simulink model "Bidirection_EVSE_V2G_and_G2V"  (R2024b)
settings: Solver=VariableStepAuto  StartTime=0.0  StopTime=10.0  RelTol=1e-3
undefined symbols (not defined in the file): Ion, Lithium
libraries: spsIdealSwitchLib x6, spsSeriesRLCBranchLib x6, slpidlib x4, spsPWMGeneratorDCDCLib x4, spsMosfetLib x4, spsVoltageMeasurementLib x4, spsThreePhaseSeriesRLCLoadLib x3, spsThreePhaseVIMeasurementLib x2, spsUniversalBridgeLib x2, spsBatteryLib x1, spsPLL3phLib x1, spsPower3phInstantaneousLib x1
settings Model: Creator=SUDHAK1  LastModifiedBy=SUDHAK1

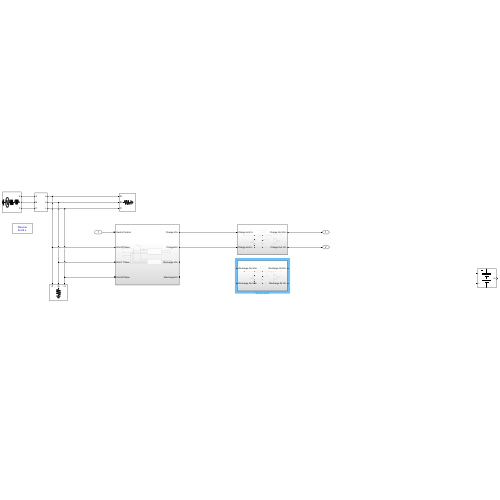
[thumbnail: Simulink's stored preview of the top-level diagram]
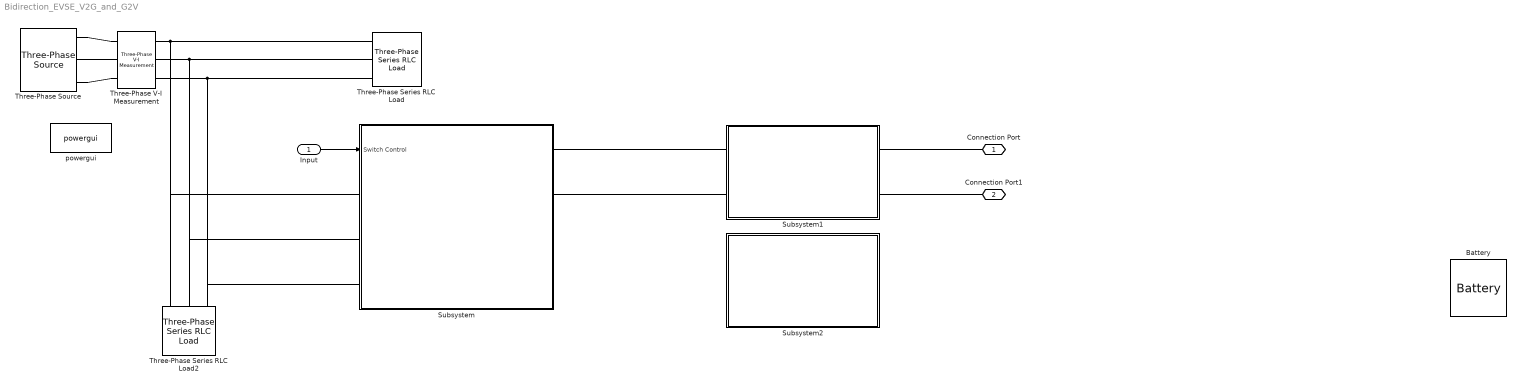
== system Bidirection_EVSE_V2G_and_G2V ==
  Input : Inport
  Battery : spsBatteryLib/Battery  BatType=Lithium-Ion  NomV=230  NomQ=100  SOC=60  Batt_Tr=1e-3  PresetModel=on  MaxQ=100  MinV=172.5  FullV=267.717  Dis_rate=43.4783  R=0.023  Normal_OP=90.4348  expZone="[248.4887      4.913043]"
  Subsystem : Subsystem
  Subsystem1 : Subsystem
  Subsystem2 : Subsystem
  Three-Phase Series RLC Load : spsThreePhaseSeriesRLCLoadLib/Three-Phase Series RLC Load  LConnTagsString=A|B|C  Configuration=Y (grounded)  NominalVoltage=380  Vabc=[1e3 1e3 1e3]  Vabcp=[1e3 1e3 1e3]  NominalFrequency=50  UnbalancedPower=off  ActivePower=10e3  InductivePower=0  CapacitivePower=0  Pabc=[10e3 9e3 11e3]  QLabc=[100 90 110]  QCabc=[100 90 110]  Pabcp=[10e3 9e3 11e3]  QLabcp=[100 90 110]  QCabcp=[100 90 110]  Measurements=None  LoadType=constant Z
  Three-Phase Series RLC Load2 : spsThreePhaseSeriesRLCLoadLib/Three-Phase Series RLC Load  LConnTagsString=A|B|C  Configuration=Y (grounded)  NominalVoltage=380  Vabc=[1e3 1e3 1e3]  Vabcp=[1e3 1e3 1e3]  NominalFrequency=50  UnbalancedPower=off  ActivePower=10e3  InductivePower=0  CapacitivePower=0  Pabc=[10e3 9e3 11e3]  QLabc=[100 90 110]  QCabc=[100 90 110]  Pabcp=[10e3 9e3 11e3]  QLabcp=[100 90 110]  QCabcp=[100 90 110]  Measurements=None  LoadType=constant Z
  Three-Phase V-I Measurement : spsThreePhaseVIMeasurementLib/Three-Phase V-I Measurement  VoltageMeasurement=phase-to-phase  SetLabelV=on  LabelV=Vabc_grid  Vpu=off  VpuLL=off  CurrentMeasurement=yes  SetLabelI=on  LabelI=Iabc_grid  Ipu=off  Pbase=100e6  Vbase=500e3  OutputType=Complex  PhasorSimulation=off  PSBequivalent=0
  Three-Phase Source : spsThreePhaseSourceLib/Three-Phase Source  InternalConnection=Yg  VoltagePhases=off  Voltage=380  PhaseAngle=0  Voltage_phases=[25e3 25e3 25e3]/sqrt(3)  PhaseAngles_phases=[0 -120 +120]  Frequency=50  NonIdealSource=on  SpecifyImpedance=on  Resistance=0.8929  Inductance=16.58e-3  ShortCircuitLevel=100e6  BaseVoltage=380  XRratio=7  BusType=swing  Pref=10e3  Qref=0  Prefabc=[10e3, 10e3, 10e3]  Qrefabc=[0, 0, 0]  Qmin=-inf  Qmax=inf
  powergui : spspowerguiLib/powergui  Priority=1  SimulationMode=Discrete  SampleTime=5e-6  frequency=60  Iterations=50  frequencyindice=60  Pbase=100e6  ErrMax=1e-4  UnitsV=kV  UnitsW=MW  buscounter=0  FunctionMessages=off  echomessages=off  EnableUseOfTLC=off  CurrentSourceSwitches=off  DisableSnubberDevices=off  DisableRonSwitches=off  DisableVfSwitches=off  DisplayEquations=off  AutomaticDiscreteSolvers=off  SolverType=Tustin/Backward Euler (TBE)  Interpol=off  ExternalGateDelay=off  methode=off  Ts=100  x0status=blocks  SPID=on  SwTol=0  HookPort=off  NonlinearTolerance=1e-4  nMaxIteration=100  ContinueOnMaxIteration=off  RestoreLinks=warning  ResistiveCurrentMeasurement=off  Frange=[0:2:500]  Ylog=off  Xlog=on  ShowGrid=off  save=off  variable=ZData  structure=0  ZoomFFT=off  StartTime=0.0  cycles=1  DisplayStyle=1  fundamental=60  FreqAxis=off  MaxFrequency=1000  frequencyindicesteady=1  RmsSteady=1  display=off
  Connection Port : PMIOPort  Side=Left
  Connection Port1 : PMIOPort  Port=2  Side=Left
  wires:
  Input/1 -> Subsystem/1(Switch Control)
  connections:
  Three-Phase Source/RConn1 -- Three-Phase V-I Measurement/LConn1
  Three-Phase Source/RConn2 -- Three-Phase V-I Measurement/LConn2
  Three-Phase Source/RConn3 -- Three-Phase V-I Measurement/LConn3
  Three-Phase Series RLC Load/LConn1 -- Three-Phase Series RLC Load2/LConn1 -- Subsystem/LConn1 -- Three-Phase V-I Measurement/RConn1
  Three-Phase Series RLC Load/LConn2 -- Three-Phase Series RLC Load2/LConn2 -- Subsystem/LConn2 -- Three-Phase V-I Measurement/RConn2
  Three-Phase Series RLC Load/LConn3 -- Three-Phase Series RLC Load2/LConn3 -- Subsystem/LConn3 -- Three-Phase V-I Measurement/RConn3
  Subsystem/RConn1 -- Subsystem1/LConn1
  Connection Port/RConn1 -- Subsystem1/RConn1
  Subsystem/RConn2 -- Subsystem1/LConn2
  Connection Port1/RConn1 -- Subsystem1/RConn2

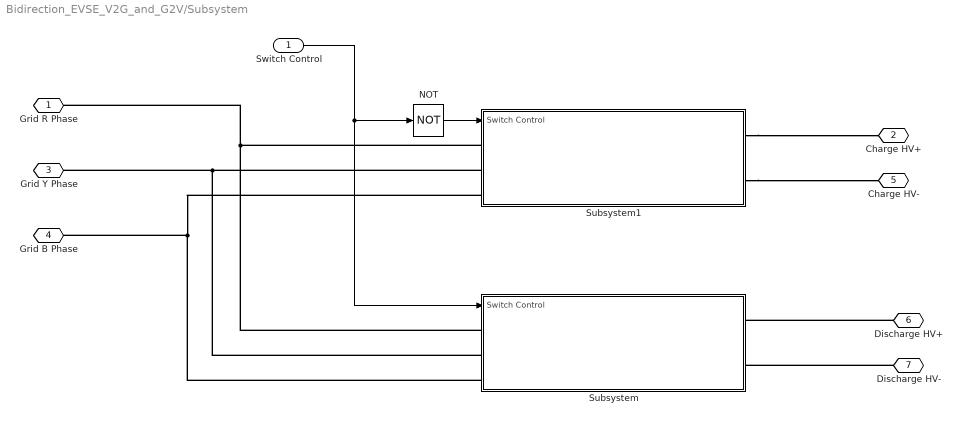
== system Bidirection_EVSE_V2G_and_G2V/Subsystem ==
  Switch Control : Inport
  NOT : Logic  Operator=NOT  IconShape=distinctive  AllPortsSameDT=off  OutDataTypeStr=boolean
  Subsystem : Subsystem
  Subsystem1 : Subsystem
  Grid R Phase : PMIOPort  Side=Left
  Charge HV+ : PMIOPort  Port=2  Side=Right
  Grid Y Phase : PMIOPort  Port=3  Side=Left
  Grid B Phase : PMIOPort  Port=4  Side=Left
  Charge HV- : PMIOPort  Port=5  Side=Right
  Discharge HV+ : PMIOPort  Port=6  Side=Right
  Discharge HV- : PMIOPort  Port=7  Side=Right
  wires:
  Switch Control/1 -> Subsystem/1(Switch Control), NOT/1
  NOT/1 -> Subsystem1/1(Switch Control)
  connections:
  Subsystem/LConn2 -- Grid Y Phase/RConn1 -- Subsystem1/LConn2
  Grid B Phase/RConn1 -- Subsystem1/LConn3 -- Subsystem/LConn3
  Subsystem/LConn1 -- Grid R Phase/RConn1 -- Subsystem1/LConn1
  Subsystem1/RConn1 -- Charge HV+/RConn1
  Subsystem1/RConn2 -- Charge HV-/RConn1
  Discharge HV-/RConn1 -- Subsystem/RConn2
  Discharge HV+/RConn1 -- Subsystem/RConn1

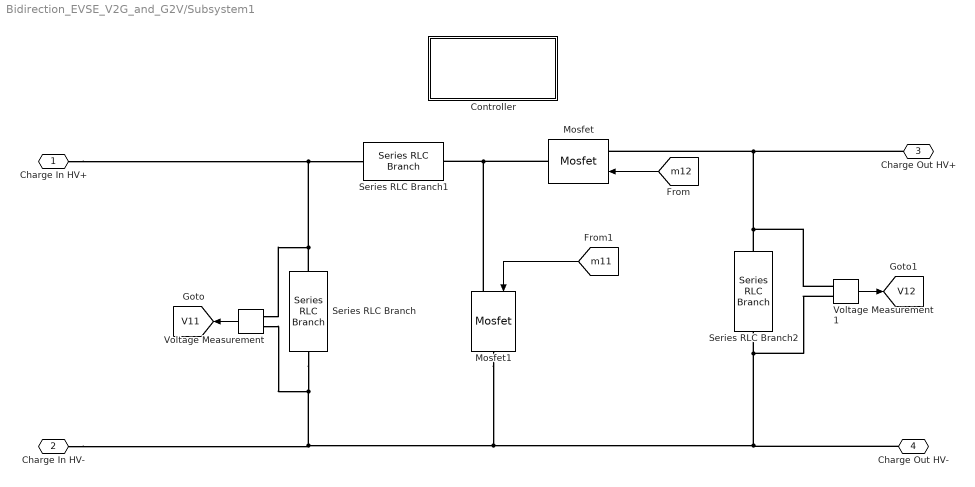
== system Bidirection_EVSE_V2G_and_G2V/Subsystem1 ==
  Controller : Subsystem
  Mosfet : spsMosfetLib/Mosfet  Ron=0.1  Lon=0  Rd=0.01  Vfd=0  IC=0  Rs=1e5  Cs=inf  Measurements=off
  Mosfet1 : spsMosfetLib/Mosfet  Ron=0.1  Lon=0  Rd=0.01  Vfd=0  IC=0  Rs=1e5  Cs=inf  Measurements=off
  Series RLC Branch : spsSeriesRLCBranchLib/Series RLC Branch  LConnTagsString=__new0  RConnTagsString=__new0  BranchType=RC  Resistance=0.0001  Inductance=1e-3  SetiL0=off  InitialCurrent=0  Capacitance=1000e-6  Setx0=off  InitialVoltage=0  Measurements=None
  Series RLC Branch1 : spsSeriesRLCBranchLib/Series RLC Branch  LConnTagsString=__new0  RConnTagsString=__new0  BranchType=L  Resistance=0.0001  Inductance=1e-3  SetiL0=off  InitialCurrent=0  Capacitance=1000e-6  Setx0=off  InitialVoltage=0  Measurements=None
  Series RLC Branch2 : spsSeriesRLCBranchLib/Series RLC Branch  LConnTagsString=__new0  RConnTagsString=__new0  BranchType=RC  Resistance=0.0001  Inductance=1e-3  SetiL0=off  InitialCurrent=0  Capacitance=1000e-6  Setx0=off  InitialVoltage=0  Measurements=None
  Voltage Measurement : spsVoltageMeasurementLib/Voltage Measurement  PhasorSimulation=off  OutputType=Complex  PSBequivalent=0
  Voltage Measurement1 : spsVoltageMeasurementLib/Voltage Measurement  PhasorSimulation=off  OutputType=Complex  PSBequivalent=0
  Charge In HV+ : PMIOPort  Side=Left
  Charge In HV- : PMIOPort  Port=2  Side=Left
  Charge Out HV+ : PMIOPort  Port=3  Side=Right
  Charge Out HV- : PMIOPort  Port=4  Side=Right
  tag scope: V11=global, V12=global
  wires:
  Voltage Measurement1/1 -> [V12]
  Voltage Measurement/1 -> [V11]
  [m11] -> Mosfet1/1
  [m12] -> Mosfet/1
  connections:
  Series RLC Branch/RConn1 -- Charge In HV-/RConn1 -- Mosfet1/RConn1 -- Charge Out HV-/RConn1 -- Voltage Measurement1/LConn2 -- Series RLC Branch2/RConn1 -- Voltage Measurement/LConn2
  Voltage Measurement/LConn1 -- Charge In HV+/RConn1 -- Series RLC Branch1/LConn1 -- Series RLC Branch/LConn1
  Series RLC Branch2/LConn1 -- Voltage Measurement1/LConn1 -- Charge Out HV+/RConn1 -- Mosfet/LConn1
  Mosfet/RConn1 -- Mosfet1/LConn1 -- Series RLC Branch1/RConn1

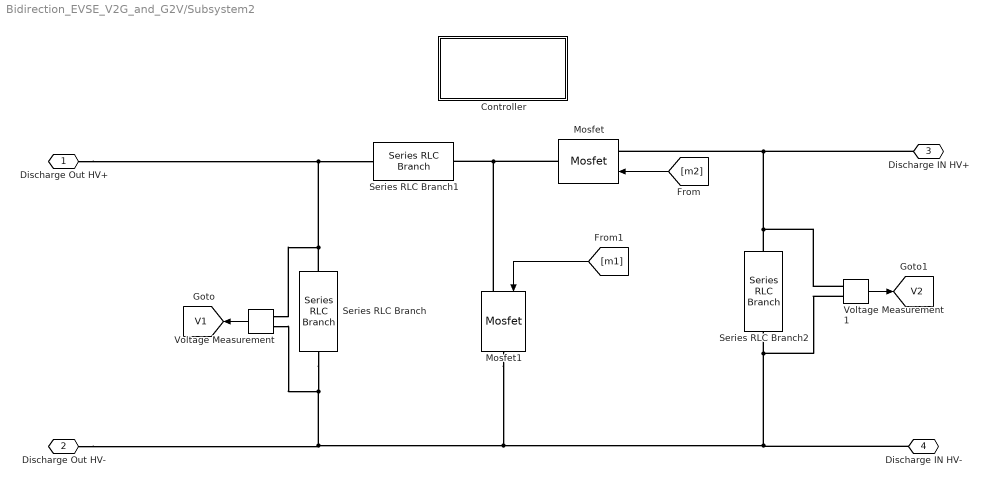
== system Bidirection_EVSE_V2G_and_G2V/Subsystem2 ==
  Controller : Subsystem
  Mosfet : spsMosfetLib/Mosfet  Ron=0.1  Lon=0  Rd=0.01  Vfd=0  IC=0  Rs=1e5  Cs=inf  Measurements=off
  Mosfet1 : spsMosfetLib/Mosfet  Ron=0.1  Lon=0  Rd=0.01  Vfd=0  IC=0  Rs=1e5  Cs=inf  Measurements=off
  Series RLC Branch : spsSeriesRLCBranchLib/Series RLC Branch  LConnTagsString=__new0  RConnTagsString=__new0  BranchType=RC  Resistance=0.0001  Inductance=1e-3  SetiL0=off  InitialCurrent=0  Capacitance=1000e-6  Setx0=off  InitialVoltage=0  Measurements=None
  Series RLC Branch1 : spsSeriesRLCBranchLib/Series RLC Branch  LConnTagsString=__new0  RConnTagsString=__new0  BranchType=L  Resistance=0.0001  Inductance=1e-3  SetiL0=off  InitialCurrent=0  Capacitance=1000e-6  Setx0=off  InitialVoltage=0  Measurements=None
  Series RLC Branch2 : spsSeriesRLCBranchLib/Series RLC Branch  LConnTagsString=__new0  RConnTagsString=__new0  BranchType=RC  Resistance=0.0001  Inductance=1e-3  SetiL0=off  InitialCurrent=0  Capacitance=1000e-6  Setx0=off  InitialVoltage=0  Measurements=None
  Voltage Measurement : spsVoltageMeasurementLib/Voltage Measurement  PhasorSimulation=off  OutputType=Complex  PSBequivalent=0
  Voltage Measurement1 : spsVoltageMeasurementLib/Voltage Measurement  PhasorSimulation=off  OutputType=Complex  PSBequivalent=0
  Discharge Out HV+ : PMIOPort  Side=Left
  Discharge Out HV- : PMIOPort  Port=2  Side=Left
  Discharge IN HV+ : PMIOPort  Port=3  Side=Right
  Discharge IN HV- : PMIOPort  Port=4  Side=Right
  tag scope: V1=global, V2=global
  wires:
  Voltage Measurement1/1 -> [V2]
  Voltage Measurement/1 -> [V1]
  [m1] -> Mosfet1/1
  [m2] -> Mosfet/1
  connections:
  Series RLC Branch/RConn1 -- Voltage Measurement/LConn2 -- Discharge Out HV-/RConn1 -- Mosfet1/RConn1 -- Discharge IN HV-/RConn1 -- Voltage Measurement1/LConn2 -- Series RLC Branch2/RConn1
  Voltage Measurement/LConn1 -- Series RLC Branch/LConn1 -- Series RLC Branch1/LConn1 -- Discharge Out HV+/RConn1
  Voltage Measurement1/LConn1 -- Series RLC Branch2/LConn1 -- Discharge IN HV+/RConn1 -- Mosfet/LConn1
  Mosfet/RConn1 -- Series RLC Branch1/RConn1 -- Mosfet1/LConn1

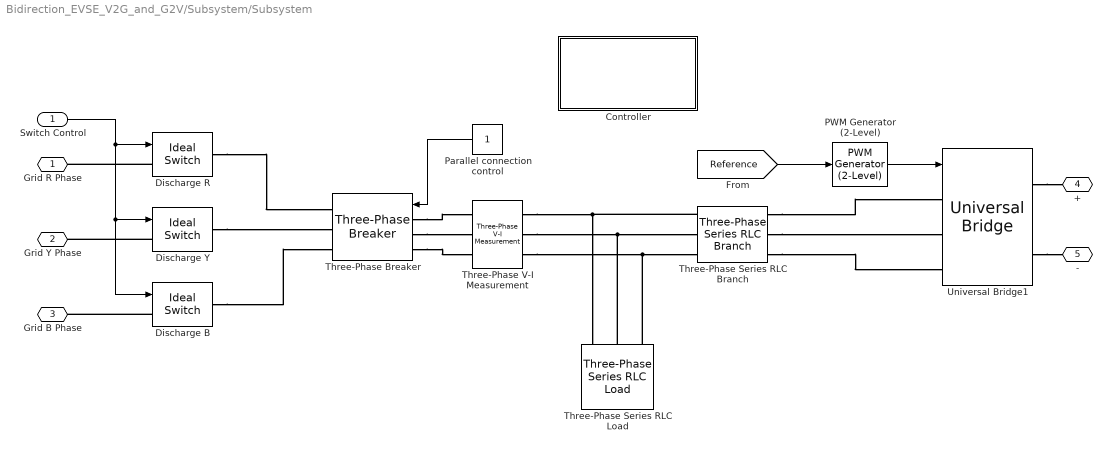
== system Bidirection_EVSE_V2G_and_G2V/Subsystem/Subsystem ==
  Switch Control : Inport
  Controller : Subsystem
  Discharge B : spsIdealSwitchLib/Ideal Switch  Ron=1e-6  Lon=0  IC=0  Rs=1e5  Cs=inf  Measurements=off
  Discharge R : spsIdealSwitchLib/Ideal Switch  Ron=1e-6  Lon=0  IC=0  Rs=1e5  Cs=inf  Measurements=off
  Discharge Y : spsIdealSwitchLib/Ideal Switch  Ron=1e-6  Lon=0  IC=0  Rs=1e5  Cs=inf  Measurements=off
  PWM Generator (2-Level) : spsPWMGenerator2LevelLib/PWM Generator (2-Level)  ModulatorType=Three-phase bridge (6 pulses)  ModulatorMode=Unsynchronized  Fc=4950  Pc=90  nF=27  MinMax="[ -1  1 ]"  SamplingTechnique=Natural  ModulatingSignals=off  m=0.8  Freq=60  Phase=0  Ts=2.02e-6  ShowCarrierOutport=off
  Parallel connection control : Constant
  Three-Phase Series RLC Branch : spsThreePhaseSeriesRLCBranchLib/Three-Phase Series RLC Branch  LConnTagsString=A|B|C  RConnTagsString=A|B|C  BranchType=RL  Resistance=0.004332  Inductance=0.0013789184  Capacitance=1e-6  Measurements=None
  Three-Phase Series RLC Load : spsThreePhaseSeriesRLCLoadLib/Three-Phase Series RLC Load  LConnTagsString=A|B|C  Configuration=Delta  NominalVoltage=380  Vabc=[1e3 1e3 1e3]  Vabcp=[1e3 1e3 1e3]  NominalFrequency=50  UnbalancedPower=off  ActivePower=100  InductivePower=0  CapacitivePower=5000  Pabc=[10e3 9e3 11e3]  QLabc=[100 90 110]  QCabc=[100 90 110]  Pabcp=[10e3 9e3 11e3]  QLabcp=[100 90 110]  QCabcp=[100 90 110]  Measurements=None  LoadType=constant Z
  Three-Phase V-I Measurement : spsThreePhaseVIMeasurementLib/Three-Phase V-I Measurement  VoltageMeasurement=phase-to-phase  SetLabelV=on  LabelV=Vabc_inv  Vpu=off  VpuLL=off  CurrentMeasurement=yes  SetLabelI=on  LabelI=Iabc_inv  Ipu=off  Pbase=100e6  Vbase=500e3  OutputType=Complex  PhasorSimulation=off  PSBequivalent=0
  Three-Phase Breaker : spsThreePhaseBreakerLib/Three-Phase Breaker  InitialState=open  SwitchA=on  SwitchB=on  SwitchC=on  SwitchTimes="[1/60  5/60]"  External=on  BreakerResistance=0.01  SnubberResistance=1e6  SnubberCapacitance=inf  Measurements=None
  Universal Bridge1 : spsUniversalBridgeLib/Universal Bridge  Arms=3  SnubberResistance=1e6  SnubberCapacitance=inf  Device=IGBT / Diodes  Ron=1e-3  Lon=0  ForwardVoltages="[  0  0  ]"  ForwardVoltage=0  GTOparameters=[ 10e-6 , 20e-6 ]  IGBTparameters=[ 1e-6 , 2e-6 ]  Measurements=None  Measurements_2=None  converterType=Rectifier
  Grid R Phase : PMIOPort  Side=Left
  Grid Y Phase : PMIOPort  Port=2  Side=Left
  Grid B Phase : PMIOPort  Port=3  Side=Left
  + : PMIOPort  Port=4  Side=Right
  - : PMIOPort  Port=5  Side=Right
  wires:
  [Reference] -> PWM Generator (2-Level)/1
  PWM Generator (2-Level)/1 -> Universal Bridge1/1
  Switch Control/1 -> Discharge B/1, Discharge Y/1, Discharge R/1
  Parallel connection control/1 -> Three-Phase Breaker/1
  connections:
  Three-Phase Series RLC Branch/LConn3 -- Universal Bridge1/LConn3
  Three-Phase Breaker/LConn1 -- Three-Phase V-I Measurement/RConn1
  Three-Phase Series RLC Branch/RConn1 -- Three-Phase Series RLC Load/LConn1 -- Three-Phase V-I Measurement/LConn1
  Three-Phase Breaker/LConn2 -- Three-Phase V-I Measurement/RConn2
  Discharge B/RConn1 -- Three-Phase Breaker/RConn3
  Discharge Y/RConn1 -- Three-Phase Breaker/RConn2
  Three-Phase Breaker/LConn3 -- Three-Phase V-I Measurement/RConn3
  Discharge R/RConn1 -- Three-Phase Breaker/RConn1
  Three-Phase Series RLC Load/LConn3 -- Three-Phase V-I Measurement/LConn3 -- Three-Phase Series RLC Branch/RConn3
  Three-Phase Series RLC Load/LConn2 -- Three-Phase V-I Measurement/LConn2 -- Three-Phase Series RLC Branch/RConn2
  Discharge B/LConn1 -- Grid B Phase/RConn1
  Three-Phase Series RLC Branch/LConn1 -- Universal Bridge1/LConn1
  Three-Phase Series RLC Branch/LConn2 -- Universal Bridge1/LConn2
  Discharge R/LConn1 -- Grid R Phase/RConn1
  Universal Bridge1/RConn2 -- -/RConn1
  Discharge Y/LConn1 -- Grid Y Phase/RConn1
  Universal Bridge1/RConn1 -- +/RConn1

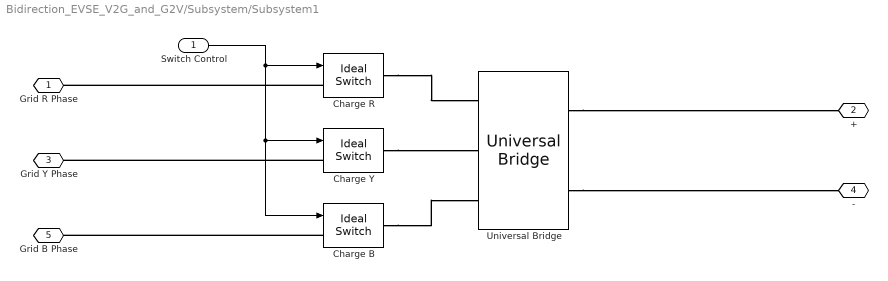
== system Bidirection_EVSE_V2G_and_G2V/Subsystem/Subsystem1 ==
  Switch Control : Inport
  Charge B : spsIdealSwitchLib/Ideal Switch  Ron=1e-6  Lon=0  IC=0  Rs=1e5  Cs=inf  Measurements=off
  Charge R : spsIdealSwitchLib/Ideal Switch  Ron=1e-6  Lon=0  IC=0  Rs=1e5  Cs=inf  Measurements=off
  Charge Y : spsIdealSwitchLib/Ideal Switch  Ron=1e-6  Lon=0  IC=0  Rs=1e5  Cs=inf  Measurements=off
  Universal Bridge : spsUniversalBridgeLib/Universal Bridge  Arms=3  SnubberResistance=1e5  SnubberCapacitance=inf  Device=Diodes  Ron=1e-3  Lon=0  ForwardVoltages="[  0  0  ]"  ForwardVoltage=0  GTOparameters=[ 10e-6 , 20e-6 ]  IGBTparameters=[ 1e-6 , 2e-6 ]  Measurements=None  Measurements_2=None  converterType=Rectifier
  Grid R Phase : PMIOPort  Side=Left
  + : PMIOPort  Port=2  Side=Right
  Grid Y Phase : PMIOPort  Port=3  Side=Left
  - : PMIOPort  Port=4  Side=Right
  Grid B Phase : PMIOPort  Port=5  Side=Left
  wires:
  Switch Control/1 -> Charge Y/1, Charge B/1, Charge R/1
  connections:
  Charge B/LConn1 -- Grid B Phase/RConn1
  Universal Bridge/RConn1 -- +/RConn1
  Charge B/RConn1 -- Universal Bridge/LConn3
  Charge R/RConn1 -- Universal Bridge/LConn1
  Charge R/LConn1 -- Grid R Phase/RConn1
  Charge Y/RConn1 -- Universal Bridge/LConn2
  Charge Y/LConn1 -- Grid Y Phase/RConn1
  Universal Bridge/RConn2 -- -/RConn1

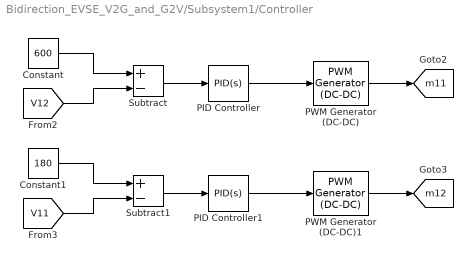
== system Bidirection_EVSE_V2G_and_G2V/Subsystem1/Controller ==
  Constant : Constant  Value=600
  Constant1 : Constant  Value=180
  PID Controller : slpidlib/PID Controller  Controller=PID  Form=Parallel  TimeDomain=Continuous-time  UseExternalTs=off  SampleTime=-1  IntegratorMethod=Forward Euler  FilterMethod=Forward Euler  ControllerParametersSource=internal  P=0  I=7  UseKiTs=off  D=0  UseExternalDerivativeSource=off  N=100  UseFilter=on  TunerSelectOption=Transfer Function Based (PID Tuner App)  InitialConditionSource=internal  InitialConditionForIntegrator=0  InitialConditionForFilter=0  DifferentiatorICPrevScaledInput=0  ExternalReset=none  TrackingMode=off  Kt=1  LimitOutput=off  SatLimitsSource=internal  UpperSaturationLimit=inf  LowerSaturationLimit=-inf  LinearizeAsGain=on  AntiWindupMode=none  Kb=1  LimitIntegrator=off  UpperIntegratorSaturationLimit=inf  LowerIntegratorSaturationLimit=-inf  POutMin=[]  POutMax=[]  IOutMin=[]  IOutMax=[]  DOutMin=[]  DOutMax=[]  NOutMin=[]  NOutMax=[]  SumOutMin=[]  SumOutMax=[]  SaturationOutMin=[]  SaturationOutMax=[]  PParamMin=[]  PParamMax=[]  IParamMin=[]  IParamMax=[]  DParamMin=[]  DParamMax=[]  NParamMin=[]  NParamMax=[]  KbParamMin=[]  KbParamMax=[]  KtParamMin=[]  KtParamMax=[]  KbOutMin=[]  KbOutMax=[]  KtOutMin=[]  KtOutMax=[]  IntegratorOutMin=[]  IntegratorOutMax=[]  FilterOutMin=[]  FilterOutMax=[]  SumI1OutMin=[]  SumI1OutMax=[]  SumI2OutMin=[]  SumI2OutMax=[]  SumI3OutMin=[]  SumI3OutMax=[]  SumI4OutMin=[]  SumI4OutMax=[]  SumDOutMin=[]  SumDOutMax=[]  DifferentiatorOutMin=[]  DifferentiatorOutMax=[]  FilterDiffOutCoefMin=[]  FilterDiffOutCoefMax=[]  ReciprocalOutMin=[]  ReciprocalOutMax=[]  SumDenOutMin=[]  SumDenOutMax=[]  SumNumOutMin=[]  SumNumOutMax=[]  DivideOutMin=[]  DivideOutMax=[]  UdiffTsProdOutMin=[]  UdiffTsProdOutMax=[]  NTsProdOutMin=[]  NTsProdOutMax=[]  UintegralTsProdOutMin=[]  UintegralTsProdOutMax=[]  UngainTsProdOutMin=[]  UngainTsProdOutMax=[]  ClampingZeroOutDataTypeStr=Inherit: Inherit via back propagation  ClampingZeroOutMin=[]  ClampingZeroOutMax=[]  FilterDenConstantOutDataTypeStr=Inherit: Inherit via back propagation  FilterDenConstantOutMin=[]  FilterDenConstantOutMax=[]  PCopyOutDataTypeStr=Inherit: Inherit via back propagation  PCopyOutMin=[]  PCopyOutMax=[]  NCopyOutDataTypeStr=Inherit: Inherit via back propagation  NCopyOutMin=[]  NCopyOutMax=[]  IntegratorContinuousStateAttributes=''  IntegratorStateMustResolveToSignalObject=off  IntegratorRTWStateStorageClass=Auto  FilterContinuousStateAttributes=''  FilterStateMustResolveToSignalObject=off  FilterRTWStateStorageClass=Auto  ParallelPVariant=InternalParameters  IdealPVariant=Disabled  IVariant=InternalParameters  DVariant=InternalParameters  IntegratorVariant=Continuous  SatVariant=Disabled  AWVariant=Passthrough  PCopyVariant=Disabled  TRVariant=Disabled  FdbkBlocksVariant=Forward  IdealPFdbkVariant=Disabled  SatFdbkVariant=Disabled  DerivativeFilterVariant=ContFilter  NVariant=InternalParameters  NCopyVariant=Disabled  FilterICVariant=InternalICsFilter  IntegratorICVariant=InternalICs  ExternalResetVariant=Disabled  TRSumVariant=Passthrough  SumFdbkVariant=Disabled  SumVariant=Sum_PID  TsampFilterVariant=InternalTs  TsampNgainVariant=Passthrough  TsampIntegralVariant=Disabled_SignalSpec  ExternalSaturationOutDataTypeStr=Inherit: Same as second input  DerivativeSourceVariant=ErrorSignal  PreIntVariant=InternalPreInt
  PID Controller1 : slpidlib/PID Controller  Controller=PID  Form=Parallel  TimeDomain=Continuous-time  UseExternalTs=off  SampleTime=-1  IntegratorMethod=Forward Euler  FilterMethod=Forward Euler  ControllerParametersSource=internal  P=0  I=7  UseKiTs=off  D=0  UseExternalDerivativeSource=off  N=100  UseFilter=on  TunerSelectOption=Transfer Function Based (PID Tuner App)  InitialConditionSource=internal  InitialConditionForIntegrator=0  InitialConditionForFilter=0  DifferentiatorICPrevScaledInput=0  ExternalReset=none  TrackingMode=off  Kt=1  LimitOutput=off  SatLimitsSource=internal  UpperSaturationLimit=inf  LowerSaturationLimit=-inf  LinearizeAsGain=on  AntiWindupMode=none  Kb=1  LimitIntegrator=off  UpperIntegratorSaturationLimit=inf  LowerIntegratorSaturationLimit=-inf  POutMin=[]  POutMax=[]  IOutMin=[]  IOutMax=[]  DOutMin=[]  DOutMax=[]  NOutMin=[]  NOutMax=[]  SumOutMin=[]  SumOutMax=[]  SaturationOutMin=[]  SaturationOutMax=[]  PParamMin=[]  PParamMax=[]  IParamMin=[]  IParamMax=[]  DParamMin=[]  DParamMax=[]  NParamMin=[]  NParamMax=[]  KbParamMin=[]  KbParamMax=[]  KtParamMin=[]  KtParamMax=[]  KbOutMin=[]  KbOutMax=[]  KtOutMin=[]  KtOutMax=[]  IntegratorOutMin=[]  IntegratorOutMax=[]  FilterOutMin=[]  FilterOutMax=[]  SumI1OutMin=[]  SumI1OutMax=[]  SumI2OutMin=[]  SumI2OutMax=[]  SumI3OutMin=[]  SumI3OutMax=[]  SumI4OutMin=[]  SumI4OutMax=[]  SumDOutMin=[]  SumDOutMax=[]  DifferentiatorOutMin=[]  DifferentiatorOutMax=[]  FilterDiffOutCoefMin=[]  FilterDiffOutCoefMax=[]  ReciprocalOutMin=[]  ReciprocalOutMax=[]  SumDenOutMin=[]  SumDenOutMax=[]  SumNumOutMin=[]  SumNumOutMax=[]  DivideOutMin=[]  DivideOutMax=[]  UdiffTsProdOutMin=[]  UdiffTsProdOutMax=[]  NTsProdOutMin=[]  NTsProdOutMax=[]  UintegralTsProdOutMin=[]  UintegralTsProdOutMax=[]  UngainTsProdOutMin=[]  UngainTsProdOutMax=[]  ClampingZeroOutDataTypeStr=Inherit: Inherit via back propagation  ClampingZeroOutMin=[]  ClampingZeroOutMax=[]  FilterDenConstantOutDataTypeStr=Inherit: Inherit via back propagation  FilterDenConstantOutMin=[]  FilterDenConstantOutMax=[]  PCopyOutDataTypeStr=Inherit: Inherit via back propagation  PCopyOutMin=[]  PCopyOutMax=[]  NCopyOutDataTypeStr=Inherit: Inherit via back propagation  NCopyOutMin=[]  NCopyOutMax=[]  IntegratorContinuousStateAttributes=''  IntegratorStateMustResolveToSignalObject=off  IntegratorRTWStateStorageClass=Auto  FilterContinuousStateAttributes=''  FilterStateMustResolveToSignalObject=off  FilterRTWStateStorageClass=Auto  ParallelPVariant=InternalParameters  IdealPVariant=Disabled  IVariant=InternalParameters  DVariant=InternalParameters  IntegratorVariant=Continuous  SatVariant=Disabled  AWVariant=Passthrough  PCopyVariant=Disabled  TRVariant=Disabled  FdbkBlocksVariant=Forward  IdealPFdbkVariant=Disabled  SatFdbkVariant=Disabled  DerivativeFilterVariant=ContFilter  NVariant=InternalParameters  NCopyVariant=Disabled  FilterICVariant=InternalICsFilter  IntegratorICVariant=InternalICs  ExternalResetVariant=Disabled  TRSumVariant=Passthrough  SumFdbkVariant=Disabled  SumVariant=Sum_PID  TsampFilterVariant=InternalTs  TsampNgainVariant=Passthrough  TsampIntegralVariant=Disabled_SignalSpec  ExternalSaturationOutDataTypeStr=Inherit: Same as second input  DerivativeSourceVariant=ErrorSignal  PreIntVariant=InternalPreInt
  PWM Generator (DC-DC) : spsPWMGeneratorDCDCLib/PWM Generator (DC-DC)  Fsw=5000  Ts=0
  PWM Generator (DC-DC)1 : spsPWMGeneratorDCDCLib/PWM Generator (DC-DC)  Fsw=5000  Ts=0
  Subtract : Sum  Inputs=+-
  Subtract1 : Sum  Inputs=+-
  tag scope: m11=global, m12=global
  wires:
  Constant/1 -> Subtract/1
  PID Controller1/1 -> PWM Generator (DC-DC)1/1
  [V11] -> Subtract1/2
  Constant1/1 -> Subtract1/1
  PWM Generator (DC-DC)1/1 -> [m12]
  [V12] -> Subtract/2
  PWM Generator (DC-DC)/1 -> [m11]
  Subtract/1 -> PID Controller/1
  Subtract1/1 -> PID Controller1/1
  PID Controller/1 -> PWM Generator (DC-DC)/1

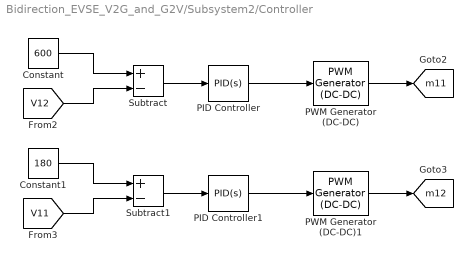
== system Bidirection_EVSE_V2G_and_G2V/Subsystem2/Controller ==
  Constant : Constant  Value=600
  Constant1 : Constant  Value=180
  PID Controller : slpidlib/PID Controller  Controller=PID  Form=Parallel  TimeDomain=Continuous-time  UseExternalTs=off  SampleTime=-1  IntegratorMethod=Forward Euler  FilterMethod=Forward Euler  ControllerParametersSource=internal  P=0  I=7  UseKiTs=off  D=0  UseExternalDerivativeSource=off  N=100  UseFilter=on  TunerSelectOption=Transfer Function Based (PID Tuner App)  InitialConditionSource=internal  InitialConditionForIntegrator=0  InitialConditionForFilter=0  DifferentiatorICPrevScaledInput=0  ExternalReset=none  TrackingMode=off  Kt=1  LimitOutput=off  SatLimitsSource=internal  UpperSaturationLimit=inf  LowerSaturationLimit=-inf  LinearizeAsGain=on  AntiWindupMode=none  Kb=1  LimitIntegrator=off  UpperIntegratorSaturationLimit=inf  LowerIntegratorSaturationLimit=-inf  POutMin=[]  POutMax=[]  IOutMin=[]  IOutMax=[]  DOutMin=[]  DOutMax=[]  NOutMin=[]  NOutMax=[]  SumOutMin=[]  SumOutMax=[]  SaturationOutMin=[]  SaturationOutMax=[]  PParamMin=[]  PParamMax=[]  IParamMin=[]  IParamMax=[]  DParamMin=[]  DParamMax=[]  NParamMin=[]  NParamMax=[]  KbParamMin=[]  KbParamMax=[]  KtParamMin=[]  KtParamMax=[]  KbOutMin=[]  KbOutMax=[]  KtOutMin=[]  KtOutMax=[]  IntegratorOutMin=[]  IntegratorOutMax=[]  FilterOutMin=[]  FilterOutMax=[]  SumI1OutMin=[]  SumI1OutMax=[]  SumI2OutMin=[]  SumI2OutMax=[]  SumI3OutMin=[]  SumI3OutMax=[]  SumI4OutMin=[]  SumI4OutMax=[]  SumDOutMin=[]  SumDOutMax=[]  DifferentiatorOutMin=[]  DifferentiatorOutMax=[]  FilterDiffOutCoefMin=[]  FilterDiffOutCoefMax=[]  ReciprocalOutMin=[]  ReciprocalOutMax=[]  SumDenOutMin=[]  SumDenOutMax=[]  SumNumOutMin=[]  SumNumOutMax=[]  DivideOutMin=[]  DivideOutMax=[]  UdiffTsProdOutMin=[]  UdiffTsProdOutMax=[]  NTsProdOutMin=[]  NTsProdOutMax=[]  UintegralTsProdOutMin=[]  UintegralTsProdOutMax=[]  UngainTsProdOutMin=[]  UngainTsProdOutMax=[]  ClampingZeroOutDataTypeStr=Inherit: Inherit via back propagation  ClampingZeroOutMin=[]  ClampingZeroOutMax=[]  FilterDenConstantOutDataTypeStr=Inherit: Inherit via back propagation  FilterDenConstantOutMin=[]  FilterDenConstantOutMax=[]  PCopyOutDataTypeStr=Inherit: Inherit via back propagation  PCopyOutMin=[]  PCopyOutMax=[]  NCopyOutDataTypeStr=Inherit: Inherit via back propagation  NCopyOutMin=[]  NCopyOutMax=[]  IntegratorContinuousStateAttributes=''  IntegratorStateMustResolveToSignalObject=off  IntegratorRTWStateStorageClass=Auto  FilterContinuousStateAttributes=''  FilterStateMustResolveToSignalObject=off  FilterRTWStateStorageClass=Auto  ParallelPVariant=InternalParameters  IdealPVariant=Disabled  IVariant=InternalParameters  DVariant=InternalParameters  IntegratorVariant=Continuous  SatVariant=Disabled  AWVariant=Passthrough  PCopyVariant=Disabled  TRVariant=Disabled  FdbkBlocksVariant=Forward  IdealPFdbkVariant=Disabled  SatFdbkVariant=Disabled  DerivativeFilterVariant=ContFilter  NVariant=InternalParameters  NCopyVariant=Disabled  FilterICVariant=InternalICsFilter  IntegratorICVariant=InternalICs  ExternalResetVariant=Disabled  TRSumVariant=Passthrough  SumFdbkVariant=Disabled  SumVariant=Sum_PID  TsampFilterVariant=InternalTs  TsampNgainVariant=Passthrough  TsampIntegralVariant=Disabled_SignalSpec  ExternalSaturationOutDataTypeStr=Inherit: Same as second input  DerivativeSourceVariant=ErrorSignal  PreIntVariant=InternalPreInt
  PID Controller1 : slpidlib/PID Controller  Controller=PID  Form=Parallel  TimeDomain=Continuous-time  UseExternalTs=off  SampleTime=-1  IntegratorMethod=Forward Euler  FilterMethod=Forward Euler  ControllerParametersSource=internal  P=0  I=7  UseKiTs=off  D=0  UseExternalDerivativeSource=off  N=100  UseFilter=on  TunerSelectOption=Transfer Function Based (PID Tuner App)  InitialConditionSource=internal  InitialConditionForIntegrator=0  InitialConditionForFilter=0  DifferentiatorICPrevScaledInput=0  ExternalReset=none  TrackingMode=off  Kt=1  LimitOutput=off  SatLimitsSource=internal  UpperSaturationLimit=inf  LowerSaturationLimit=-inf  LinearizeAsGain=on  AntiWindupMode=none  Kb=1  LimitIntegrator=off  UpperIntegratorSaturationLimit=inf  LowerIntegratorSaturationLimit=-inf  POutMin=[]  POutMax=[]  IOutMin=[]  IOutMax=[]  DOutMin=[]  DOutMax=[]  NOutMin=[]  NOutMax=[]  SumOutMin=[]  SumOutMax=[]  SaturationOutMin=[]  SaturationOutMax=[]  PParamMin=[]  PParamMax=[]  IParamMin=[]  IParamMax=[]  DParamMin=[]  DParamMax=[]  NParamMin=[]  NParamMax=[]  KbParamMin=[]  KbParamMax=[]  KtParamMin=[]  KtParamMax=[]  KbOutMin=[]  KbOutMax=[]  KtOutMin=[]  KtOutMax=[]  IntegratorOutMin=[]  IntegratorOutMax=[]  FilterOutMin=[]  FilterOutMax=[]  SumI1OutMin=[]  SumI1OutMax=[]  SumI2OutMin=[]  SumI2OutMax=[]  SumI3OutMin=[]  SumI3OutMax=[]  SumI4OutMin=[]  SumI4OutMax=[]  SumDOutMin=[]  SumDOutMax=[]  DifferentiatorOutMin=[]  DifferentiatorOutMax=[]  FilterDiffOutCoefMin=[]  FilterDiffOutCoefMax=[]  ReciprocalOutMin=[]  ReciprocalOutMax=[]  SumDenOutMin=[]  SumDenOutMax=[]  SumNumOutMin=[]  SumNumOutMax=[]  DivideOutMin=[]  DivideOutMax=[]  UdiffTsProdOutMin=[]  UdiffTsProdOutMax=[]  NTsProdOutMin=[]  NTsProdOutMax=[]  UintegralTsProdOutMin=[]  UintegralTsProdOutMax=[]  UngainTsProdOutMin=[]  UngainTsProdOutMax=[]  ClampingZeroOutDataTypeStr=Inherit: Inherit via back propagation  ClampingZeroOutMin=[]  ClampingZeroOutMax=[]  FilterDenConstantOutDataTypeStr=Inherit: Inherit via back propagation  FilterDenConstantOutMin=[]  FilterDenConstantOutMax=[]  PCopyOutDataTypeStr=Inherit: Inherit via back propagation  PCopyOutMin=[]  PCopyOutMax=[]  NCopyOutDataTypeStr=Inherit: Inherit via back propagation  NCopyOutMin=[]  NCopyOutMax=[]  IntegratorContinuousStateAttributes=''  IntegratorStateMustResolveToSignalObject=off  IntegratorRTWStateStorageClass=Auto  FilterContinuousStateAttributes=''  FilterStateMustResolveToSignalObject=off  FilterRTWStateStorageClass=Auto  ParallelPVariant=InternalParameters  IdealPVariant=Disabled  IVariant=InternalParameters  DVariant=InternalParameters  IntegratorVariant=Continuous  SatVariant=Disabled  AWVariant=Passthrough  PCopyVariant=Disabled  TRVariant=Disabled  FdbkBlocksVariant=Forward  IdealPFdbkVariant=Disabled  SatFdbkVariant=Disabled  DerivativeFilterVariant=ContFilter  NVariant=InternalParameters  NCopyVariant=Disabled  FilterICVariant=InternalICsFilter  IntegratorICVariant=InternalICs  ExternalResetVariant=Disabled  TRSumVariant=Passthrough  SumFdbkVariant=Disabled  SumVariant=Sum_PID  TsampFilterVariant=InternalTs  TsampNgainVariant=Passthrough  TsampIntegralVariant=Disabled_SignalSpec  ExternalSaturationOutDataTypeStr=Inherit: Same as second input  DerivativeSourceVariant=ErrorSignal  PreIntVariant=InternalPreInt
  PWM Generator (DC-DC) : spsPWMGeneratorDCDCLib/PWM Generator (DC-DC)  Fsw=5000  Ts=0
  PWM Generator (DC-DC)1 : spsPWMGeneratorDCDCLib/PWM Generator (DC-DC)  Fsw=5000  Ts=0
  Subtract : Sum  Inputs=+-
  Subtract1 : Sum  Inputs=+-
  tag scope: m11=global, m12=global
  wires:
  Constant/1 -> Subtract/1
  PID Controller1/1 -> PWM Generator (DC-DC)1/1
  [V11] -> Subtract1/2
  Constant1/1 -> Subtract1/1
  PWM Generator (DC-DC)1/1 -> [m12]
  [V12] -> Subtract/2
  PWM Generator (DC-DC)/1 -> [m11]
  Subtract/1 -> PID Controller/1
  Subtract1/1 -> PID Controller1/1
  PID Controller/1 -> PWM Generator (DC-DC)/1

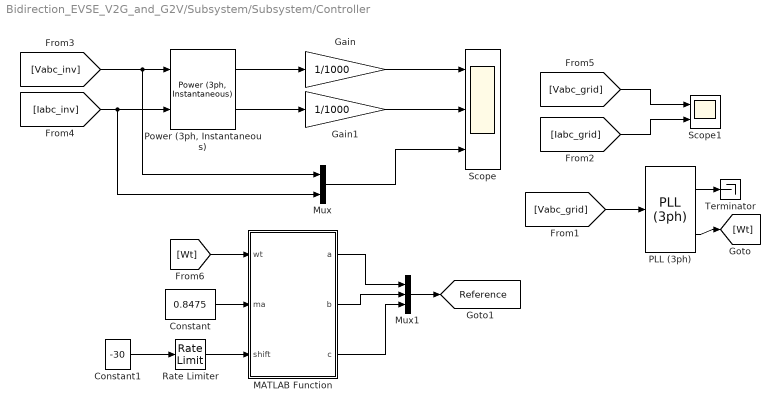
== system Bidirection_EVSE_V2G_and_G2V/Subsystem/Subsystem/Controller ==
  Constant : Constant  Value=0.8475
  Constant1 : Constant  Value=-30
  Gain : Gain  Gain=1/1000
  Gain1 : Gain  Gain=1/1000
  MATLAB Function : MATLAB Function  TreatAsAtomicUnit=on
  Mux : Mux  Inputs=2
  Mux1 : Mux  Inputs=3
  PLL (3ph) : spsPLL3phLib/PLL (3ph)  Fmin=45  Par_Init=[0, 50]  ParK=[180, 3200, 1]  TcD=1e-4  MaxRateChangeFreq=12  FilterCutOffFreq=25  Ts=0  AGC=on
  "Power (3ph, Instantaneous)" : spsPower3phInstantaneousLib/Power (3ph, Instantaneous)
  Rate Limiter : RateLimiter  SampleTimeMode=inherited
  Scope : Scope  NumInputPorts=3
  Scope1 : Scope  NumInputPorts=2
  Terminator : Terminator
  tag scope: Reference=global
  wires:
  [Vabc_inv] -> Mux/1, "Power (3ph, Instantaneous)"/1
  [Iabc_grid] -> Scope1/2
  Constant/1 -> MATLAB Function/2(ma)
  [Wt] -> MATLAB Function/1(wt)
  Gain/1 -> Scope/1
  Gain1/1 -> Scope/2
  [Vabc_grid] -> Scope1/1
  MATLAB Function/2(b) -> Mux1/2
  MATLAB Function/1(a) -> Mux1/1
  "Power (3ph, Instantaneous)"/1 -> Gain/1
  [Iabc_inv] -> "Power (3ph, Instantaneous)"/2, Mux/2
  Rate Limiter/1 -> MATLAB Function/3(shift)
  [Vabc_grid] -> PLL (3ph)/1
  Constant1/1 -> Rate Limiter/1
  PLL (3ph)/2 -> [Wt]
  MATLAB Function/3(c) -> Mux1/3
  Mux1/1 -> [Reference]
  Mux/1 -> Scope/3
  "Power (3ph, Instantaneous)"/2 -> Gain1/1
  PLL (3ph)/1 -> Terminator/1

== matlab function Bidirection_EVSE_V2G_and_G2V/Subsystem/Subsystem/Controller/MATLAB Function ==
  data: wt input; a output; ma input; shift input; b output; c output
function [a,b,c] = fcn(wt,ma,shift)

shift_k=shift*pi/180;
a = (ma*(sin((x)+shift_k)));
b = (ma*(sin((x)+shift_k-(2*pi/3))));
c = (ma*(sin((x)+shift_k+(2*pi/3))));
